simulink model "PCS261S_Original_Temperature_Control_Model"  (R2026a)
settings: Solver=VariableStepAuto  StopTime=1500
libraries: simulink x1
settings Model: Creator=nnete  LastModifiedBy=nnete

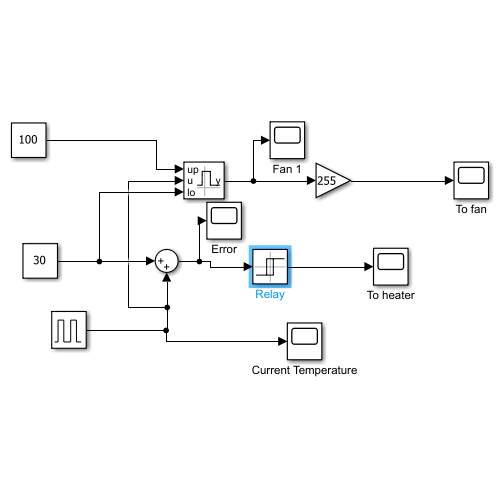
[thumbnail: Simulink's stored preview of the top-level diagram]
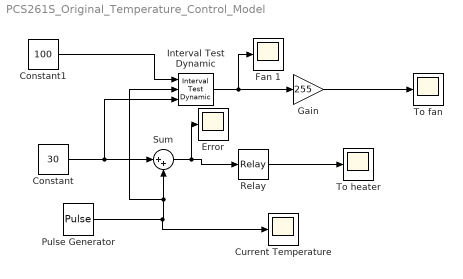
== system PCS261S_Original_Temperature_Control_Model ==
  Constant : Constant  Value=30
  Constant1 : Constant  Value=100
  Current Temperature : Scope
      settings: DataLoggingVariableName=ScopeData2
  Error : Scope
      settings: ActiveDisplayYMinimum=26.25  ActiveDisplayYMaximum=63.75  DataLoggingVariableName=ScopeData4
  Fan 1 : Scope
      settings: ActiveDisplayYMinimum=-0.12499999999999997  ActiveDisplayYMaximum=1.125  DataLoggingVariableName=ScopeData3
  Gain : Gain  Gain=255
  Interval Test Dynamic : simulink/Logic and Bit Operations/Interval Test Dynamic  IntervalClosedRight=on  IntervalClosedLeft=on  OutDataTypeStr=boolean
  Pulse Generator : DiscretePulseGenerator  PulseType=Time based  Amplitude=30  Period=180  PulseWidth=50
  Relay : Relay  OnSwitchValue=0.1  OffSwitchValue=0.0001  OnOutputValue=255
  Sum : Sum  Inputs=|++
  To fan : Scope
      settings: ActiveDisplayYMinimum=-31.874999999999993  ActiveDisplayYMaximum=286.875
  To heater : Scope
      settings: ActiveDisplayYMinimum=134.32043143915655  ActiveDisplayYMaximum=381.0589734850326
  wires:
  Pulse Generator/1 -> Current Temperature/1, Interval Test Dynamic/2, Sum/2
  Constant/1 -> Interval Test Dynamic/3, Sum/1
  Sum/1 -> Error/1, Relay/1
  Relay/1 -> To heater/1
  Constant1/1 -> Interval Test Dynamic/1
  Interval Test Dynamic/1 -> Fan 1/1, Gain/1
  Gain/1 -> To fan/1
